simulink model "DCX_Facility"  (R2024a)
settings: Solver=FixedStepDiscrete  StartTime=0.0  StopTime=3600  FixedStep=1  RelTol=1e-3
PreLoadFcn:
  | dcx_model_data();
values from neighbouring files (symbols this model uses):
  CMD = struct('seq',0,'code',0,'asset',0,'value',0)    [dcx_model_data.m]
  P = evalin('base', 'P')    [dcx_build_model.m]
  SP = P.sp    [dcx_model_data.m]
undefined symbols (not defined in the file or in its folder): ats_ats_s, ats_cooldown_s, ats_gen_start_s, ats_retransfer_s, BRIDGE, X0, Y0
libraries: slpidlib x7
settings Model: Creator=deshm  LastModifiedBy=deshm
settings DebuggingCC: AlgebraicLoopMsg=error  UnconnectedInputMsg=error

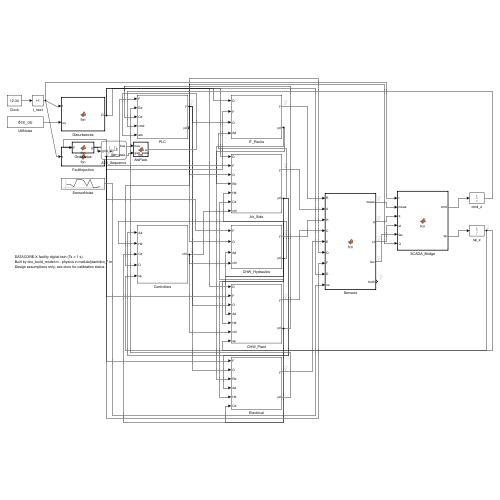
[thumbnail: Simulink's stored preview of the top-level diagram]
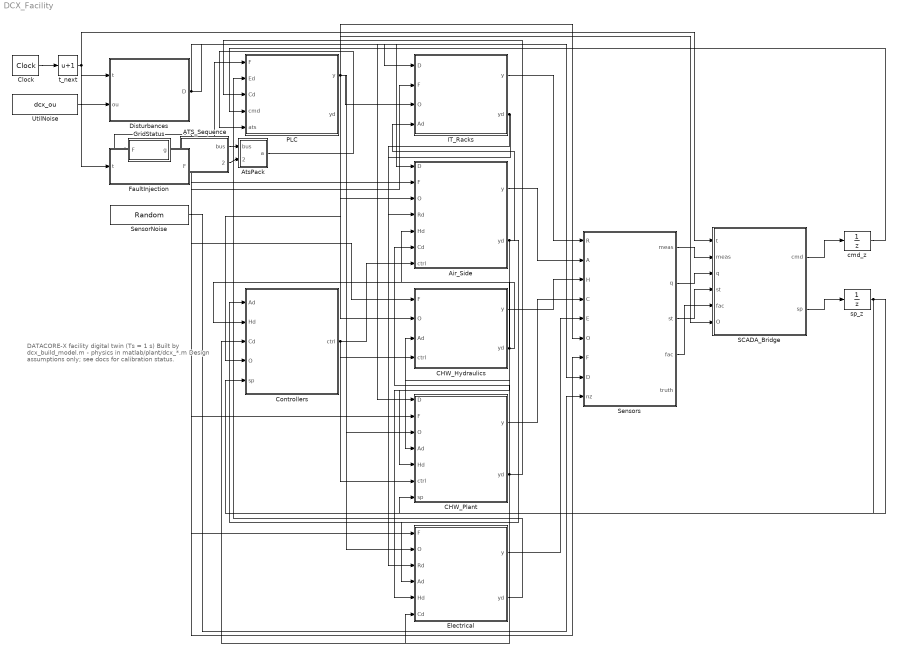
== system DCX_Facility ==
  note: DATACORE-X facility digital twin (Ts = 1 s)
      | Built by dcx_build_model.m - physics in matlab/plant/dcx_*.m
      | Design assumptions only; see docs for calibration status.
  ATS_Sequence : Stateflow chart  TreatAsAtomicUnit=on
  Air_Side : Subsystem
  AtsPack : MATLAB Function  TreatAsAtomicUnit=on
  CHW_Hydraulics : Subsystem
  CHW_Plant : Subsystem
  Clock : DigitalClock
  Controllers : Subsystem
  Disturbances : MATLAB Function  TreatAsAtomicUnit=on
  Electrical : Subsystem
  FaultInjection : MATLAB Function  TreatAsAtomicUnit=on
  GridStatus : MATLAB Function  TreatAsAtomicUnit=on
  IT_Racks : Subsystem
  PLC : Subsystem
  SCADA_Bridge : MATLAB Function  TreatAsAtomicUnit=on
  SensorNoise : RandomNumber  Mean=zeros(1,217)  Seed=P.seed + 4 + (1:217)  SampleTime=1
  Sensors : MATLAB Function  TreatAsAtomicUnit=on
  UtilNoise : FromWorkspace  VariableName=dcx_ou  SampleTime=1  Interpolate=off  OutputAfterFinalValue=Holding final value
  cmd_z : UnitDelay  InitialCondition=CMD  HasFrameUpgradeWarning=on
  sp_z : UnitDelay  InitialCondition=SP  HasFrameUpgradeWarning=on
  t_next : Bias  Bias=1  SaturateOnIntegerOverflow=off
  wires:
  Clock/1 -> t_next/1
  t_next/1 -> Disturbances/1(t), FaultInjection/1(t), SCADA_Bridge/1(t)
  UtilNoise/1 -> Disturbances/2(ou)
  FaultInjection/1(F) -> PLC/1(F), GridStatus/1(F), IT_Racks/2(F), Air_Side/2(F), CHW_Hydraulics/1(F), CHW_Plant/2(F), Electrical/1(F), Sensors/7(F)
  Electrical/2(yd) -> PLC/2(Ed)
  CHW_Plant/2(yd) -> PLC/3(Cd), Air_Side/6(Cd), Electrical/6(Cd), Controllers/3(Cd)
  cmd_z/1 -> PLC/4(cmd)
  GridStatus/1(g) -> ATS_Sequence/1(grid_ok)
  ATS_Sequence/1(bus) -> AtsPack/1(bus)
  ATS_Sequence/2(gen_state) -> AtsPack/2(gen_state)
  AtsPack/1(a) -> PLC/5(ats)
  Disturbances/1(D) -> IT_Racks/1(D), Air_Side/1(D), CHW_Plant/1(D), Sensors/8(D)
  PLC/1(y) -> IT_Racks/3(O), Air_Side/3(O), CHW_Hydraulics/2(O), CHW_Plant/3(O), Electrical/2(O), Controllers/4(O), Sensors/6(O), SCADA_Bridge/6(O)
  Air_Side/2(yd) -> IT_Racks/4(Ad), CHW_Hydraulics/3(Ad), CHW_Plant/4(Ad), Electrical/4(Ad), Controllers/1(Ad)
  IT_Racks/2(yd) -> Air_Side/4(Rd), Electrical/3(Rd)
  CHW_Hydraulics/2(yd) -> Air_Side/5(Hd), CHW_Plant/5(Hd), Electrical/5(Hd), Controllers/2(Hd)
  Controllers/1(ctrl) -> Air_Side/7(ctrl), CHW_Hydraulics/4(ctrl), CHW_Plant/6(ctrl)
  sp_z/1 -> CHW_Plant/7(sp), Controllers/5(sp)
  IT_Racks/1(y) -> Sensors/1(R)
  Air_Side/1(y) -> Sensors/2(A)
  CHW_Hydraulics/1(y) -> Sensors/3(H)
  CHW_Plant/1(y) -> Sensors/4(C)
  Electrical/1(y) -> Sensors/5(E)
  SensorNoise/1 -> Sensors/9(nz)
  Sensors/1(meas) -> SCADA_Bridge/2(meas)
  Sensors/2(q) -> SCADA_Bridge/3(q)
  Sensors/3(st) -> SCADA_Bridge/4(st)
  Sensors/4(fac) -> SCADA_Bridge/5(fac)
  SCADA_Bridge/1(cmd) -> cmd_z/1
  SCADA_Bridge/2(sp) -> sp_z/1

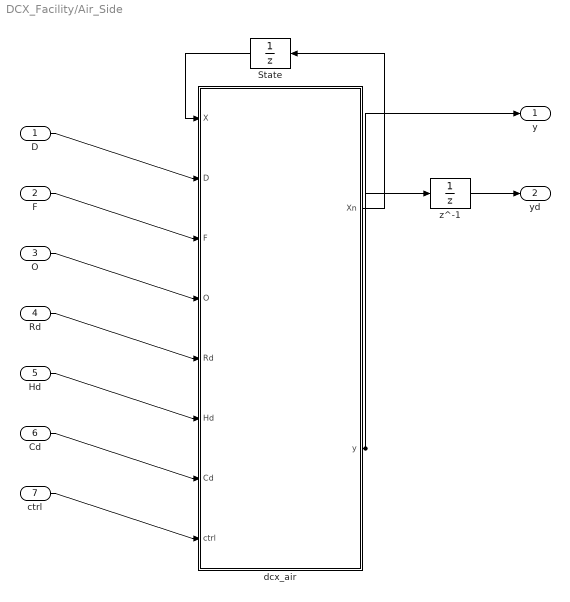
== system DCX_Facility/Air_Side ==
  D : Inport
  F : Inport  Port=2
  O : Inport  Port=3
  Rd : Inport  Port=4
  Hd : Inport  Port=5
  Cd : Inport  Port=6
  ctrl : Inport  Port=7
  State : UnitDelay  InitialCondition=X0.air  HasFrameUpgradeWarning=on
  dcx_air : MATLAB Function  TreatAsAtomicUnit=on
  z^-1 : UnitDelay  InitialCondition=Y0.A  HasFrameUpgradeWarning=on
  y : Outport
  yd : Outport  Port=2
  wires:
  dcx_air/1(Xn) -> State/1
  State/1 -> dcx_air/1(X)
  D/1 -> dcx_air/2(D)
  F/1 -> dcx_air/3(F)
  O/1 -> dcx_air/4(O)
  Rd/1 -> dcx_air/5(Rd)
  Hd/1 -> dcx_air/6(Hd)
  Cd/1 -> dcx_air/7(Cd)
  ctrl/1 -> dcx_air/8(ctrl)
  dcx_air/2(y) -> y/1, z^-1/1
  z^-1/1 -> yd/1

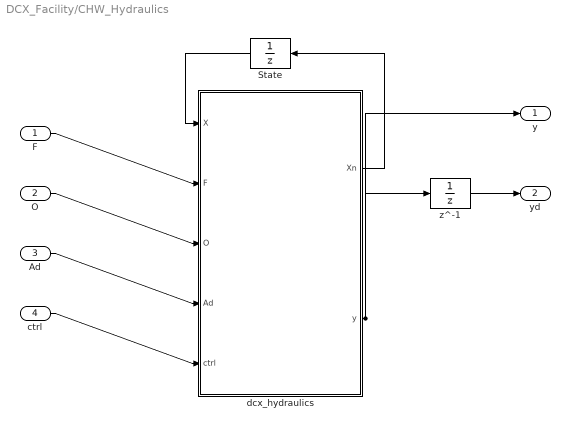
== system DCX_Facility/CHW_Hydraulics ==
  F : Inport
  O : Inport  Port=2
  Ad : Inport  Port=3
  ctrl : Inport  Port=4
  State : UnitDelay  InitialCondition=X0.hyd  HasFrameUpgradeWarning=on
  dcx_hydraulics : MATLAB Function  TreatAsAtomicUnit=on
  z^-1 : UnitDelay  InitialCondition=Y0.H  HasFrameUpgradeWarning=on
  y : Outport
  yd : Outport  Port=2
  wires:
  dcx_hydraulics/1(Xn) -> State/1
  State/1 -> dcx_hydraulics/1(X)
  F/1 -> dcx_hydraulics/2(F)
  O/1 -> dcx_hydraulics/3(O)
  Ad/1 -> dcx_hydraulics/4(Ad)
  ctrl/1 -> dcx_hydraulics/5(ctrl)
  dcx_hydraulics/2(y) -> y/1, z^-1/1
  z^-1/1 -> yd/1

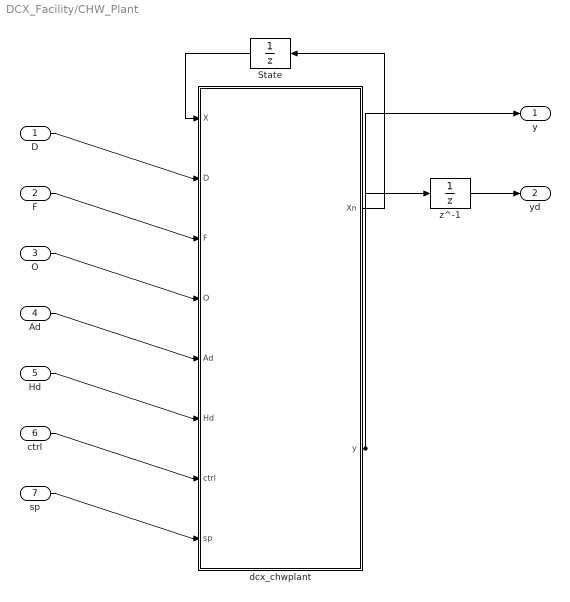
== system DCX_Facility/CHW_Plant ==
  D : Inport
  F : Inport  Port=2
  O : Inport  Port=3
  Ad : Inport  Port=4
  Hd : Inport  Port=5
  ctrl : Inport  Port=6
  sp : Inport  Port=7
  State : UnitDelay  InitialCondition=X0.chw  HasFrameUpgradeWarning=on
  dcx_chwplant : MATLAB Function  TreatAsAtomicUnit=on
  z^-1 : UnitDelay  InitialCondition=Y0.C  HasFrameUpgradeWarning=on
  y : Outport
  yd : Outport  Port=2
  wires:
  dcx_chwplant/1(Xn) -> State/1
  State/1 -> dcx_chwplant/1(X)
  D/1 -> dcx_chwplant/2(D)
  F/1 -> dcx_chwplant/3(F)
  O/1 -> dcx_chwplant/4(O)
  Ad/1 -> dcx_chwplant/5(Ad)
  Hd/1 -> dcx_chwplant/6(Hd)
  ctrl/1 -> dcx_chwplant/7(ctrl)
  sp/1 -> dcx_chwplant/8(sp)
  dcx_chwplant/2(y) -> y/1, z^-1/1
  z^-1/1 -> yd/1

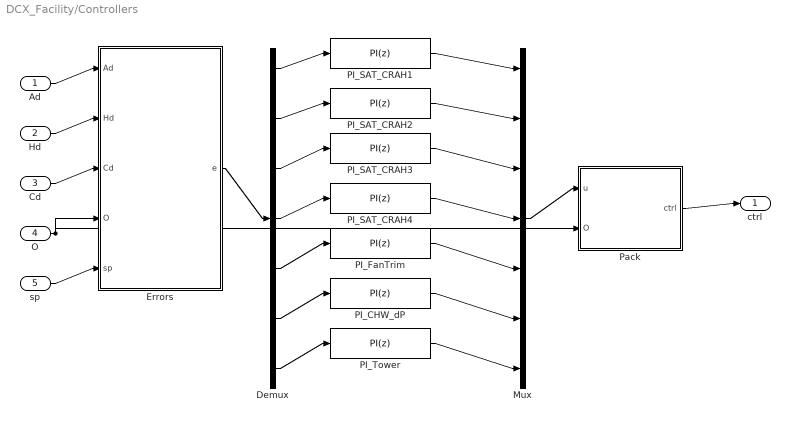
== system DCX_Facility/Controllers ==
  Ad : Inport
  Hd : Inport  Port=2
  Cd : Inport  Port=3
  O : Inport  Port=4
  sp : Inport  Port=5
  Demux : Demux  Outputs=7
  Errors : MATLAB Function  TreatAsAtomicUnit=on
  Mux : Mux  Inputs=7
  PI_CHW_dP : slpidlib/PID Controller  Controller=PI  Form=Parallel  TimeDomain=Discrete-time  UseExternalTs=off  SampleTime=1  IntegratorMethod=Forward Euler  FilterMethod=Forward Euler  ControllerParametersSource=internal  P=0.001  I=0.0002  UseKiTs=off  D=0  UseExternalDerivativeSource=off  N=100  UseFilter=on  TunerSelectOption=Transfer Function Based (PID Tuner App)  InitialConditionSource=internal  InitialConditionForIntegrator=0.75  InitialConditionForFilter=0  DifferentiatorICPrevScaledInput=0  ExternalReset=none  TrackingMode=off  Kt=1  LimitOutput=on  SatLimitsSource=internal  UpperSaturationLimit=1  LowerSaturationLimit=0.3  LinearizeAsGain=off  AntiWindupMode=clamping  Kb=1  LimitIntegrator=off  UpperIntegratorSaturationLimit=inf  LowerIntegratorSaturationLimit=-inf  POutMin=[]  POutMax=[]  IOutMin=[]  IOutMax=[]  DOutMin=[]  DOutMax=[]  NOutMin=[]  NOutMax=[]  SumOutMin=[]  SumOutMax=[]  SaturationOutMin=[]  SaturationOutMax=[]  PParamMin=[]  PParamMax=[]  IParamMin=[]  IParamMax=[]  DParamMin=[]  DParamMax=[]  NParamMin=[]  NParamMax=[]  KbParamMin=[]  KbParamMax=[]  KtParamMin=[]  KtParamMax=[]  KbOutMin=[]  KbOutMax=[]  KtOutMin=[]  KtOutMax=[]  IntegratorOutMin=[]  IntegratorOutMax=[]  FilterOutMin=[]  FilterOutMax=[]  SumI1OutMin=[]  SumI1OutMax=[]  SumI2OutMin=[]  SumI2OutMax=[]  SumI3OutMin=[]  SumI3OutMax=[]  SumI4OutMin=[]  SumI4OutMax=[]  SumDOutMin=[]  SumDOutMax=[]  DifferentiatorOutMin=[]  DifferentiatorOutMax=[]  FilterDiffOutCoefMin=[]  FilterDiffOutCoefMax=[]  ReciprocalOutMin=[]  ReciprocalOutMax=[]  SumDenOutMin=[]  SumDenOutMax=[]  SumNumOutMin=[]  SumNumOutMax=[]  DivideOutMin=[]  DivideOutMax=[]  UdiffTsProdOutMin=[]  UdiffTsProdOutMax=[]  NTsProdOutMin=[]  NTsProdOutMax=[]  UintegralTsProdOutMin=[]  UintegralTsProdOutMax=[]  UngainTsProdOutMin=[]  UngainTsProdOutMax=[]  ClampingZeroOutDataTypeStr=Inherit: Inherit via back propagation  ClampingZeroOutMin=[]  ClampingZeroOutMax=[]  FilterDenConstantOutDataTypeStr=Inherit: Inherit via back propagation  FilterDenConstantOutMin=[]  FilterDenConstantOutMax=[]  PCopyOutDataTypeStr=Inherit: Inherit via back propagation  PCopyOutMin=[]  PCopyOutMax=[]  NCopyOutDataTypeStr=Inherit: Inherit via back propagation  NCopyOutMin=[]  NCopyOutMax=[]  IntegratorContinuousStateAttributes=''  IntegratorStateMustResolveToSignalObject=off  IntegratorRTWStateStorageClass=Auto  FilterContinuousStateAttributes=''  FilterStateMustResolveToSignalObject=off  FilterRTWStateStorageClass=Auto  ParallelPVariant=InternalParameters  IdealPVariant=Disabled  IVariant=InternalParameters  DVariant=Disabled  IntegratorVariant=Discrete  SatVariant=Enabled  AWVariant=DiscClampingParallel  PCopyVariant=Disabled  TRVariant=Disabled  FdbkBlocksVariant=Forward  IdealPFdbkVariant=Disabled  SatFdbkVariant=Disabled  DerivativeFilterVariant=Disabled  NVariant=Disabled  NCopyVariant=Disabled_SignalSpec  FilterICVariant=Disabled  IntegratorICVariant=InternalICs  ExternalResetVariant=Disabled  TRSumVariant=Passthrough  SumFdbkVariant=Disabled  SumVariant=Sum_PI  TsampFilterVariant=InternalTs  TsampNgainVariant=Passthrough  TsampIntegralVariant=Disabled_SignalSpec  ExternalSaturationOutDataTypeStr=Inherit: Same as second input  DerivativeSourceVariant=Disabled
      settings: LibrarySourceBlock=simulink/Discrete/Discrete PID Controller
  PI_FanTrim : slpidlib/PID Controller  Controller=PI  Form=Parallel  TimeDomain=Discrete-time  UseExternalTs=off  SampleTime=1  IntegratorMethod=Forward Euler  FilterMethod=Forward Euler  ControllerParametersSource=internal  P=0.05  I=0.002  UseKiTs=off  D=0  UseExternalDerivativeSource=off  N=100  UseFilter=on  TunerSelectOption=Transfer Function Based (PID Tuner App)  InitialConditionSource=internal  InitialConditionForIntegrator=0  InitialConditionForFilter=0  DifferentiatorICPrevScaledInput=0  ExternalReset=none  TrackingMode=off  Kt=1  LimitOutput=on  SatLimitsSource=internal  UpperSaturationLimit=0.5  LowerSaturationLimit=-0.3  LinearizeAsGain=off  AntiWindupMode=clamping  Kb=1  LimitIntegrator=off  UpperIntegratorSaturationLimit=inf  LowerIntegratorSaturationLimit=-inf  POutMin=[]  POutMax=[]  IOutMin=[]  IOutMax=[]  DOutMin=[]  DOutMax=[]  NOutMin=[]  NOutMax=[]  SumOutMin=[]  SumOutMax=[]  SaturationOutMin=[]  SaturationOutMax=[]  PParamMin=[]  PParamMax=[]  IParamMin=[]  IParamMax=[]  DParamMin=[]  DParamMax=[]  NParamMin=[]  NParamMax=[]  KbParamMin=[]  KbParamMax=[]  KtParamMin=[]  KtParamMax=[]  KbOutMin=[]  KbOutMax=[]  KtOutMin=[]  KtOutMax=[]  IntegratorOutMin=[]  IntegratorOutMax=[]  FilterOutMin=[]  FilterOutMax=[]  SumI1OutMin=[]  SumI1OutMax=[]  SumI2OutMin=[]  SumI2OutMax=[]  SumI3OutMin=[]  SumI3OutMax=[]  SumI4OutMin=[]  SumI4OutMax=[]  SumDOutMin=[]  SumDOutMax=[]  DifferentiatorOutMin=[]  DifferentiatorOutMax=[]  FilterDiffOutCoefMin=[]  FilterDiffOutCoefMax=[]  ReciprocalOutMin=[]  ReciprocalOutMax=[]  SumDenOutMin=[]  SumDenOutMax=[]  SumNumOutMin=[]  SumNumOutMax=[]  DivideOutMin=[]  DivideOutMax=[]  UdiffTsProdOutMin=[]  UdiffTsProdOutMax=[]  NTsProdOutMin=[]  NTsProdOutMax=[]  UintegralTsProdOutMin=[]  UintegralTsProdOutMax=[]  UngainTsProdOutMin=[]  UngainTsProdOutMax=[]  ClampingZeroOutDataTypeStr=Inherit: Inherit via back propagation  ClampingZeroOutMin=[]  ClampingZeroOutMax=[]  FilterDenConstantOutDataTypeStr=Inherit: Inherit via back propagation  FilterDenConstantOutMin=[]  FilterDenConstantOutMax=[]  PCopyOutDataTypeStr=Inherit: Inherit via back propagation  PCopyOutMin=[]  PCopyOutMax=[]  NCopyOutDataTypeStr=Inherit: Inherit via back propagation  NCopyOutMin=[]  NCopyOutMax=[]  IntegratorContinuousStateAttributes=''  IntegratorStateMustResolveToSignalObject=off  IntegratorRTWStateStorageClass=Auto  FilterContinuousStateAttributes=''  FilterStateMustResolveToSignalObject=off  FilterRTWStateStorageClass=Auto  ParallelPVariant=InternalParameters  IdealPVariant=Disabled  IVariant=InternalParameters  DVariant=Disabled  IntegratorVariant=Discrete  SatVariant=Enabled  AWVariant=DiscClampingParallel  PCopyVariant=Disabled  TRVariant=Disabled  FdbkBlocksVariant=Forward  IdealPFdbkVariant=Disabled  SatFdbkVariant=Disabled  DerivativeFilterVariant=Disabled  NVariant=Disabled  NCopyVariant=Disabled_SignalSpec  FilterICVariant=Disabled  IntegratorICVariant=InternalICs  ExternalResetVariant=Disabled  TRSumVariant=Passthrough  SumFdbkVariant=Disabled  SumVariant=Sum_PI  TsampFilterVariant=InternalTs  TsampNgainVariant=Passthrough  TsampIntegralVariant=Disabled_SignalSpec  ExternalSaturationOutDataTypeStr=Inherit: Same as second input  DerivativeSourceVariant=Disabled
      settings: LibrarySourceBlock=simulink/Discrete/Discrete PID Controller
  PI_SAT_CRAH{1..4} (4 alike) : slpidlib/PID Controller  Controller=PI  Form=Parallel  TimeDomain=Discrete-time  UseExternalTs=off  SampleTime=1  IntegratorMethod=Forward Euler  FilterMethod=Forward Euler  ControllerParametersSource=internal  P=0.05  I=0.004  UseKiTs=off  D=0  UseExternalDerivativeSource=off  N=100  UseFilter=on  TunerSelectOption=Transfer Function Based (PID Tuner App)  InitialConditionSource=internal  InitialConditionForIntegrator=0.6  InitialConditionForFilter=0  DifferentiatorICPrevScaledInput=0  ExternalReset=none  TrackingMode=off  Kt=1  LimitOutput=on  SatLimitsSource=internal  UpperSaturationLimit=1  LowerSaturationLimit=0.05  LinearizeAsGain=off  AntiWindupMode=clamping  Kb=1  LimitIntegrator=off  UpperIntegratorSaturationLimit=inf  LowerIntegratorSaturationLimit=-inf  POutMin=[]  POutMax=[]  IOutMin=[]  IOutMax=[]  DOutMin=[]  DOutMax=[]  NOutMin=[]  NOutMax=[]  SumOutMin=[]  SumOutMax=[]  SaturationOutMin=[]  SaturationOutMax=[]  PParamMin=[]  PParamMax=[]  IParamMin=[]  IParamMax=[]  DParamMin=[]  DParamMax=[]  NParamMin=[]  NParamMax=[]  KbParamMin=[]  KbParamMax=[]  KtParamMin=[]  KtParamMax=[]  KbOutMin=[]  KbOutMax=[]  KtOutMin=[]  KtOutMax=[]  IntegratorOutMin=[]  IntegratorOutMax=[]  FilterOutMin=[]  FilterOutMax=[]  SumI1OutMin=[]  SumI1OutMax=[]  SumI2OutMin=[]  SumI2OutMax=[]  SumI3OutMin=[]  SumI3OutMax=[]  SumI4OutMin=[]  SumI4OutMax=[]  SumDOutMin=[]  SumDOutMax=[]  DifferentiatorOutMin=[]  DifferentiatorOutMax=[]  FilterDiffOutCoefMin=[]  FilterDiffOutCoefMax=[]  ReciprocalOutMin=[]  ReciprocalOutMax=[]  SumDenOutMin=[]  SumDenOutMax=[]  SumNumOutMin=[]  SumNumOutMax=[]  DivideOutMin=[]  DivideOutMax=[]  UdiffTsProdOutMin=[]  UdiffTsProdOutMax=[]  NTsProdOutMin=[]  NTsProdOutMax=[]  UintegralTsProdOutMin=[]  UintegralTsProdOutMax=[]  UngainTsProdOutMin=[]  UngainTsProdOutMax=[]  ClampingZeroOutDataTypeStr=Inherit: Inherit via back propagation  ClampingZeroOutMin=[]  ClampingZeroOutMax=[]  FilterDenConstantOutDataTypeStr=Inherit: Inherit via back propagation  FilterDenConstantOutMin=[]  FilterDenConstantOutMax=[]  PCopyOutDataTypeStr=Inherit: Inherit via back propagation  PCopyOutMin=[]  PCopyOutMax=[]  NCopyOutDataTypeStr=Inherit: Inherit via back propagation  NCopyOutMin=[]  NCopyOutMax=[]  IntegratorContinuousStateAttributes=''  IntegratorStateMustResolveToSignalObject=off  IntegratorRTWStateStorageClass=Auto  FilterContinuousStateAttributes=''  FilterStateMustResolveToSignalObject=off  FilterRTWStateStorageClass=Auto  ParallelPVariant=InternalParameters  IdealPVariant=Disabled  IVariant=InternalParameters  DVariant=Disabled  IntegratorVariant=Discrete  SatVariant=Enabled  AWVariant=DiscClampingParallel  PCopyVariant=Disabled  TRVariant=Disabled  FdbkBlocksVariant=Forward  IdealPFdbkVariant=Disabled  SatFdbkVariant=Disabled  DerivativeFilterVariant=Disabled  NVariant=Disabled  NCopyVariant=Disabled_SignalSpec  FilterICVariant=Disabled  IntegratorICVariant=InternalICs  ExternalResetVariant=Disabled  TRSumVariant=Passthrough  SumFdbkVariant=Disabled  SumVariant=Sum_PI  TsampFilterVariant=InternalTs  TsampNgainVariant=Passthrough  TsampIntegralVariant=Disabled_SignalSpec  ExternalSaturationOutDataTypeStr=Inherit: Same as second input  DerivativeSourceVariant=Disabled
      settings: LibrarySourceBlock=simulink/Discrete/Discrete PID Controller
  PI_Tower : slpidlib/PID Controller  Controller=PI  Form=Parallel  TimeDomain=Discrete-time  UseExternalTs=off  SampleTime=1  IntegratorMethod=Forward Euler  FilterMethod=Forward Euler  ControllerParametersSource=internal  P=0.12  I=0.004  UseKiTs=off  D=0  UseExternalDerivativeSource=off  N=100  UseFilter=on  TunerSelectOption=Transfer Function Based (PID Tuner App)  InitialConditionSource=internal  InitialConditionForIntegrator=0.5  InitialConditionForFilter=0  DifferentiatorICPrevScaledInput=0  ExternalReset=none  TrackingMode=off  Kt=1  LimitOutput=on  SatLimitsSource=internal  UpperSaturationLimit=1  LowerSaturationLimit=0  LinearizeAsGain=off  AntiWindupMode=clamping  Kb=1  LimitIntegrator=off  UpperIntegratorSaturationLimit=inf  LowerIntegratorSaturationLimit=-inf  POutMin=[]  POutMax=[]  IOutMin=[]  IOutMax=[]  DOutMin=[]  DOutMax=[]  NOutMin=[]  NOutMax=[]  SumOutMin=[]  SumOutMax=[]  SaturationOutMin=[]  SaturationOutMax=[]  PParamMin=[]  PParamMax=[]  IParamMin=[]  IParamMax=[]  DParamMin=[]  DParamMax=[]  NParamMin=[]  NParamMax=[]  KbParamMin=[]  KbParamMax=[]  KtParamMin=[]  KtParamMax=[]  KbOutMin=[]  KbOutMax=[]  KtOutMin=[]  KtOutMax=[]  IntegratorOutMin=[]  IntegratorOutMax=[]  FilterOutMin=[]  FilterOutMax=[]  SumI1OutMin=[]  SumI1OutMax=[]  SumI2OutMin=[]  SumI2OutMax=[]  SumI3OutMin=[]  SumI3OutMax=[]  SumI4OutMin=[]  SumI4OutMax=[]  SumDOutMin=[]  SumDOutMax=[]  DifferentiatorOutMin=[]  DifferentiatorOutMax=[]  FilterDiffOutCoefMin=[]  FilterDiffOutCoefMax=[]  ReciprocalOutMin=[]  ReciprocalOutMax=[]  SumDenOutMin=[]  SumDenOutMax=[]  SumNumOutMin=[]  SumNumOutMax=[]  DivideOutMin=[]  DivideOutMax=[]  UdiffTsProdOutMin=[]  UdiffTsProdOutMax=[]  NTsProdOutMin=[]  NTsProdOutMax=[]  UintegralTsProdOutMin=[]  UintegralTsProdOutMax=[]  UngainTsProdOutMin=[]  UngainTsProdOutMax=[]  ClampingZeroOutDataTypeStr=Inherit: Inherit via back propagation  ClampingZeroOutMin=[]  ClampingZeroOutMax=[]  FilterDenConstantOutDataTypeStr=Inherit: Inherit via back propagation  FilterDenConstantOutMin=[]  FilterDenConstantOutMax=[]  PCopyOutDataTypeStr=Inherit: Inherit via back propagation  PCopyOutMin=[]  PCopyOutMax=[]  NCopyOutDataTypeStr=Inherit: Inherit via back propagation  NCopyOutMin=[]  NCopyOutMax=[]  IntegratorContinuousStateAttributes=''  IntegratorStateMustResolveToSignalObject=off  IntegratorRTWStateStorageClass=Auto  FilterContinuousStateAttributes=''  FilterStateMustResolveToSignalObject=off  FilterRTWStateStorageClass=Auto  ParallelPVariant=InternalParameters  IdealPVariant=Disabled  IVariant=InternalParameters  DVariant=Disabled  IntegratorVariant=Discrete  SatVariant=Enabled  AWVariant=DiscClampingParallel  PCopyVariant=Disabled  TRVariant=Disabled  FdbkBlocksVariant=Forward  IdealPFdbkVariant=Disabled  SatFdbkVariant=Disabled  DerivativeFilterVariant=Disabled  NVariant=Disabled  NCopyVariant=Disabled_SignalSpec  FilterICVariant=Disabled  IntegratorICVariant=InternalICs  ExternalResetVariant=Disabled  TRSumVariant=Passthrough  SumFdbkVariant=Disabled  SumVariant=Sum_PI  TsampFilterVariant=InternalTs  TsampNgainVariant=Passthrough  TsampIntegralVariant=Disabled_SignalSpec  ExternalSaturationOutDataTypeStr=Inherit: Same as second input  DerivativeSourceVariant=Disabled
      settings: LibrarySourceBlock=simulink/Discrete/Discrete PID Controller
  Pack : MATLAB Function  TreatAsAtomicUnit=on
  ctrl : Outport
  wires:
  Ad/1 -> Errors/1(Ad)
  Hd/1 -> Errors/2(Hd)
  Cd/1 -> Errors/3(Cd)
  O/1 -> Errors/4(O), Pack/2(O)
  sp/1 -> Errors/5(sp)
  Errors/1(e) -> Demux/1
  Demux/1 -> PI_SAT_CRAH1/1
  PI_SAT_CRAH1/1 -> Mux/1
  Demux/2 -> PI_SAT_CRAH2/1
  PI_SAT_CRAH2/1 -> Mux/2
  Demux/3 -> PI_SAT_CRAH3/1
  PI_SAT_CRAH3/1 -> Mux/3
  Demux/4 -> PI_SAT_CRAH4/1
  PI_SAT_CRAH4/1 -> Mux/4
  Demux/5 -> PI_FanTrim/1
  PI_FanTrim/1 -> Mux/5
  Demux/6 -> PI_CHW_dP/1
  PI_CHW_dP/1 -> Mux/6
  Demux/7 -> PI_Tower/1
  PI_Tower/1 -> Mux/7
  Mux/1 -> Pack/1(u)
  Pack/1(ctrl) -> ctrl/1

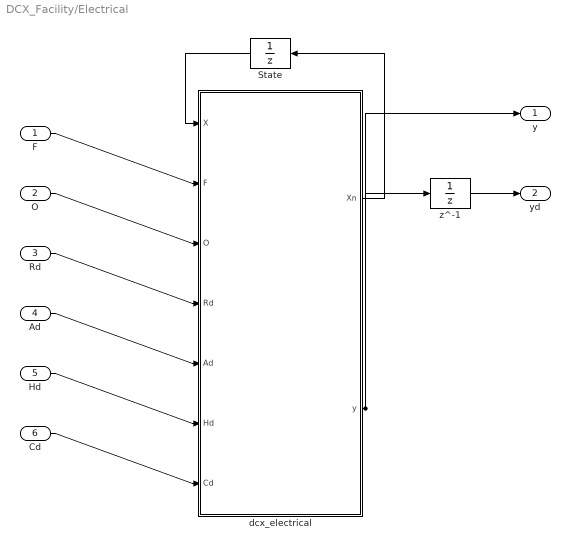
== system DCX_Facility/Electrical ==
  F : Inport
  O : Inport  Port=2
  Rd : Inport  Port=3
  Ad : Inport  Port=4
  Hd : Inport  Port=5
  Cd : Inport  Port=6
  State : UnitDelay  InitialCondition=X0.elec  HasFrameUpgradeWarning=on
  dcx_electrical : MATLAB Function  TreatAsAtomicUnit=on
  z^-1 : UnitDelay  InitialCondition=Y0.E  HasFrameUpgradeWarning=on
  y : Outport
  yd : Outport  Port=2
  wires:
  dcx_electrical/1(Xn) -> State/1
  State/1 -> dcx_electrical/1(X)
  F/1 -> dcx_electrical/2(F)
  O/1 -> dcx_electrical/3(O)
  Rd/1 -> dcx_electrical/4(Rd)
  Ad/1 -> dcx_electrical/5(Ad)
  Hd/1 -> dcx_electrical/6(Hd)
  Cd/1 -> dcx_electrical/7(Cd)
  dcx_electrical/2(y) -> y/1, z^-1/1
  z^-1/1 -> yd/1

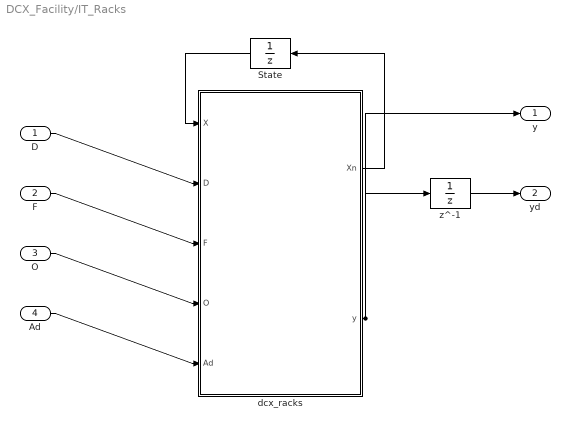
== system DCX_Facility/IT_Racks ==
  D : Inport
  F : Inport  Port=2
  O : Inport  Port=3
  Ad : Inport  Port=4
  State : UnitDelay  InitialCondition=X0.rack  HasFrameUpgradeWarning=on
  dcx_racks : MATLAB Function  TreatAsAtomicUnit=on
  z^-1 : UnitDelay  InitialCondition=Y0.R  HasFrameUpgradeWarning=on
  y : Outport
  yd : Outport  Port=2
  wires:
  dcx_racks/1(Xn) -> State/1
  State/1 -> dcx_racks/1(X)
  D/1 -> dcx_racks/2(D)
  F/1 -> dcx_racks/3(F)
  O/1 -> dcx_racks/4(O)
  Ad/1 -> dcx_racks/5(Ad)
  dcx_racks/2(y) -> y/1, z^-1/1
  z^-1/1 -> yd/1

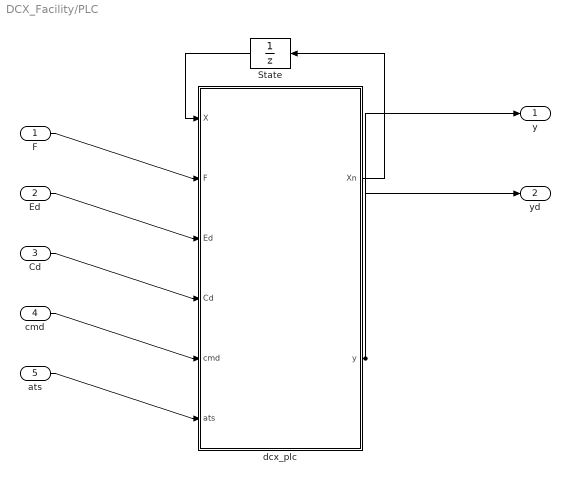
== system DCX_Facility/PLC ==
  F : Inport
  Ed : Inport  Port=2
  Cd : Inport  Port=3
  cmd : Inport  Port=4
  ats : Inport  Port=5
  State : UnitDelay  InitialCondition=X0.plc  HasFrameUpgradeWarning=on
  dcx_plc : MATLAB Function  TreatAsAtomicUnit=on
  y : Outport
  yd : Outport  Port=2
  wires:
  dcx_plc/1(Xn) -> State/1
  State/1 -> dcx_plc/1(X)
  F/1 -> dcx_plc/2(F)
  Ed/1 -> dcx_plc/3(Ed)
  Cd/1 -> dcx_plc/4(Cd)
  cmd/1 -> dcx_plc/5(cmd)
  ats/1 -> dcx_plc/6(ats)
  dcx_plc/2(y) -> y/1, yd/1

== matlab function DCX_Facility/PLC/dcx_plc ==
  data: Xn output Bus: PlcStateBus; X input; y output Bus: PlcOutBus; F input; Ed input; Cd input; cmd input; ats input; P parameter
function [Xn, y] = fcn(X, F, Ed, Cd, cmd, ats, P)
[Xn, y] = dcx_plc(X, F, Ed.soc/100, Cd.plr, cmd, P, ats);

== matlab function DCX_Facility/IT_Racks/dcx_racks ==
  data: Xn output Bus: RackStateBus; X input; y output Bus: RackBus; D input; F input; O input; Ad input; P parameter
function [Xn, y] = fcn(X, D, F, O, Ad, P)
[Xn, y] = dcx_racks(X, D, F, O, Ad, P);

== matlab function DCX_Facility/Air_Side/dcx_air ==
  data: Xn output Bus: AirStateBus; X input; y output Bus: AirBus; D input; F input; O input; Rd input; Hd input; Cd input; ctrl input; P parameter
function [Xn, y] = fcn(X, D, F, O, Rd, Hd, Cd, ctrl, P)
[Xn, y] = dcx_air(X, D, F, O, Rd, Hd, Cd, ctrl, P);

== matlab function DCX_Facility/CHW_Hydraulics/dcx_hydraulics ==
  data: Xn output Bus: HydStateBus; X input; y output Bus: HydBus; F input; O input; Ad input; ctrl input; P parameter
function [Xn, y] = fcn(X, F, O, Ad, ctrl, P)
[Xn, y] = dcx_hydraulics(X, F, O, Ad, ctrl, P);

== matlab function DCX_Facility/CHW_Plant/dcx_chwplant ==
  data: Xn output Bus: ChwStateBus; X input; y output Bus: ChwBus; D input; F input; O input; Ad input; Hd input; ctrl input; sp input; P parameter
function [Xn, y] = fcn(X, D, F, O, Ad, Hd, ctrl, sp, P)
[Xn, y] = dcx_chwplant(X, D, F, O, Ad, Hd, ctrl, sp, P);

== matlab function DCX_Facility/Electrical/dcx_electrical ==
  data: Xn output Bus: ElecStateBus; X input; y output Bus: ElecBus; F input; O input; Rd input; Ad input; Hd input; Cd input; P parameter
function [Xn, y] = fcn(X, F, O, Rd, Ad, Hd, Cd, P)
[Xn, y] = dcx_electrical(X, F, O, Rd, Ad, Hd, Cd, P);

== matlab function DCX_Facility/Controllers/Errors ==
  data: Ad input; e output size=[1 7]; Hd input; Cd input; O input; sp input
function e = fcn(Ad, Hd, Cd, O, sp)
% control errors: 4x CRAH supply air, fan trim (max inlet), CHW dP, tower leaving
e = [Ad.Tsup - sp.supply_air_c, Ad.max_in - sp.max_inlet_c, sp.dp_kpa - Hd.H, Cd.Tctl - sp.tower_leaving_c];

== matlab function DCX_Facility/Controllers/Pack ==
  data: u input size=7; ctrl output Bus: CtrlBus; O input
function ctrl = fcn(u, O)
tw = u(7); if ~any(O.tower_run > 0), tw = 0; end
ctrl = struct('fan_trim', u(5), 'valve_cmd', reshape(u(1:4),1,4), 'pump_cmd', u(6), 'tower_cmd', tw);

== matlab function DCX_Facility/Sensors ==
  data: R input; meas output size=[1 217]; A input; H input; C input; E input; O input; F input; D input; nz input; q output size=[1 217]; st output size=[1 34]; fac output size=[1 11]; truth output size=[1 217]
function [meas, q, st, fac, truth] = fcn(R, A, H, C, E, O, F, D, nz)
[meas, q, st, fac, truth] = dcx_sensors(R, A, H, C, E, O, F, D, nz);

== matlab function DCX_Facility/SCADA_Bridge ==
  data: t input; cmd output Bus: CmdBus; meas input; q input; st input; fac input; O input; sp output Bus: SpBus; CMD parameter; SP parameter; BRIDGE parameter
function [cmd, sp] = fcn(t, meas, q, st, fac, O, CMD, SP, BRIDGE)
% Simulink <-> DATACORE-X integration service (enable with BRIDGE = 1)
coder.extrinsic('dcx_bridge_tick');
cmd = CMD; sp = SP;
if BRIDGE > 0
    [cmd, sp] = dcx_bridge_tick(t, meas, q, st, fac, [O.ack_seq O.ack_code], CMD, SP);
end

== matlab function DCX_Facility/FaultInjection ==
  data: t input; F output Bus: FaultBus; FT parameter
function F = fcn(t, FT)
F = dcx_faults(t, FT);

== matlab function DCX_Facility/Disturbances ==
  data: t input; D output Bus: DistBus; ou input; P parameter
function D = fcn(t, ou, P)
D = dcx_disturbance(t, ou, P);

== matlab function DCX_Facility/GridStatus ==
  data: F input; g output
function g = fcn(F)
g = double(F.utility <= 0);

== stateflow chart DCX_Facility/ATS_Sequence ==
  settings: updateMethod=DISCRETE  sampleTime=1
  state Generator [parallel]
    settings: executionOrder=1
    state STOPPED
      entry: gen_state = 0;
    state STARTING
      entry: gen_state = 1;
    state RUNNING
      entry: gen_state = 2;
    state COOLDOWN
      entry: gen_state = 3;
    (default) -> STOPPED
    STOPPED -> STARTING : [grid_ok == 0]
    STARTING -> RUNNING [order 2] : [after(ats_gen_start_s - 1, tick)]
    STARTING -> STOPPED [order 1] : [grid_ok ~= 0]
    COOLDOWN -> STOPPED [order 2] : [after(ats_cooldown_s - 1, tick)]
    COOLDOWN -> STARTING [order 1] : [grid_ok == 0]
    RUNNING -> COOLDOWN : [grid_ok ~= 0 && in(ATS.RETRANSFER) && rt + 1 >= ats_retransfer_s]
  state ATS [parallel]
    settings: executionOrder=2
    state UTIL
      entry: bus = 1;
    state DEAD
      entry: bus = 0;
    state WAIT
      entry: bus = 0;
    state RETRANSFER
      entry: bus = 2; rt = 1;
      during: rt = rt + 1;
    state GEN
      entry: bus = 2;
    WAIT -> UTIL [order 1] : [grid_ok ~= 0]
    (default) -> UTIL
    UTIL -> DEAD : [grid_ok == 0]
    DEAD -> WAIT [order 2] : [in(Generator.RUNNING)]
    DEAD -> UTIL [order 1] : [grid_ok ~= 0]
    RETRANSFER -> UTIL [order 2] : [rt + 1 >= ats_retransfer_s]
    WAIT -> GEN [order 2] : [after(ats_ats_s - 1, tick)]
    GEN -> RETRANSFER : [grid_ok ~= 0]
    RETRANSFER -> GEN [order 1] : [grid_ok == 0]
  data: grid_ok input double; bus output double =1; gen_state output double =0; rt local double =0; ats_gen_start_s parameter double; ats_ats_s parameter double; ats_retransfer_s parameter double; ats_cooldown_s parameter double

== matlab function DCX_Facility/AtsPack ==
  data: bus input; a output; gen_state input
function a = fcn(bus, gen_state)
a = [1 bus gen_state];
